simulink model "ModelPWMGenerators"  (R2026a)
settings: Solver=VariableStepAuto  StopTime=2e-4  MaxStep=1e-7
libraries: ConverterLibrary x6
settings Model: Creator=vsolaise  LastModifiedBy=vsolaise

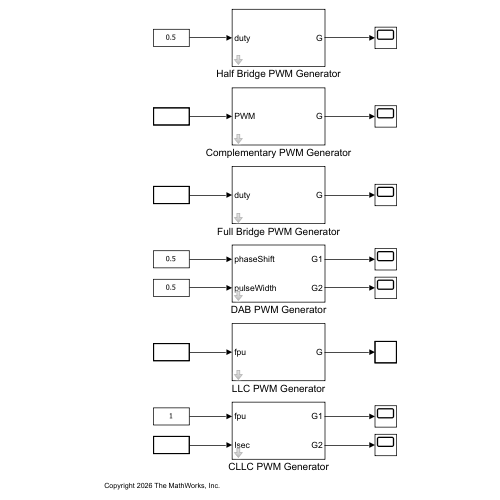
[thumbnail: Simulink's stored preview of the top-level diagram]
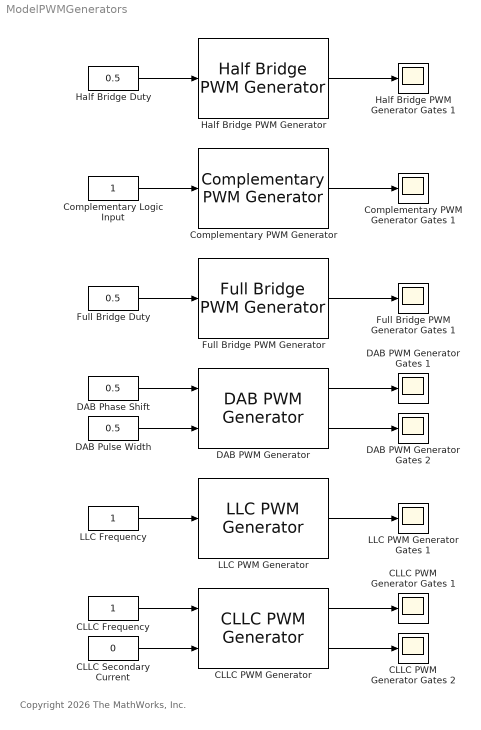
== system ModelPWMGenerators ==
  note: Copyright 2026 The MathWorks, Inc.
  CLLC Frequency : Constant
  CLLC PWM Generator : ConverterLibrary/Controller/PWM Generators/CLLC PWM Generator  solverMode=Variable-step (continuous)  Ts=1e-8  Fbase=100e3  fpuMin=0.6  fpuMax=1.55  pulseWidth=0.5  Tdead=250e-9  Ith=0.5  fpuSrLower=0.97  fpuSrUpper=1.03  Tsr=100e-9  gateVoltageOn=15  gateVoltageOff=0  srGateVoltageOn=15  srGateVoltageOff=0
  CLLC PWM Generator Gates 1 : Scope
  CLLC PWM Generator Gates 2 : Scope
  CLLC Secondary Current : Constant  Value=0
  Complementary Logic Input : Constant
  Complementary PWM Generator : ConverterLibrary/Controller/PWM Generators/Complementary PWM Generator  solverMode=Variable-step (continuous)  Ts=1e-8  Tdead=100e-9  inputLogicThreshold=0.5  gateVoltageOn=15  gateVoltageOff=0
  Complementary PWM Generator Gates 1 : Scope
  DAB PWM Generator : ConverterLibrary/Controller/PWM Generators/DAB PWM Generator  solverMode=Variable-step (continuous)  Ts=1e-8  Fsw=100e3  Tdead=100e-9  primaryGateVoltageOn=15  primaryGateVoltageOff=0  secondaryGateVoltageOn=15  secondaryGateVoltageOff=0
  DAB PWM Generator Gates 1 : Scope
  DAB PWM Generator Gates 2 : Scope
  DAB Phase Shift : Constant  Value=0.5
  DAB Pulse Width : Constant  Value=0.5
  Full Bridge Duty : Constant  Value=0.5
  Full Bridge PWM Generator : ConverterLibrary/Controller/PWM Generators/Full Bridge PWM Generator  solverMode=Variable-step (continuous)  Ts=1e-8  Fsw=100e3  Tdead=100e-9  gateVoltageOn=15  gateVoltageOff=0
  Full Bridge PWM Generator Gates 1 : Scope
  Half Bridge Duty : Constant  Value=0.5
  Half Bridge PWM Generator : ConverterLibrary/Controller/PWM Generators/Half Bridge PWM Generator  solverMode=Variable-step (continuous)  Ts=1e-8  Fsw=100e3  Tdead=100e-9  gateVoltageOn=15  gateVoltageOff=0
  Half Bridge PWM Generator Gates 1 : Scope
  LLC Frequency : Constant
  LLC PWM Generator : ConverterLibrary/Controller/PWM Generators/LLC PWM Generator  solverMode=Variable-step (continuous)  Ts=1e-8  Fbase=100e3  fpuMin=0.5  fpuMax=2  pulseWidth=0.5  Tdead=100e-9  gateVoltageOn=15  gateVoltageOff=0
  LLC PWM Generator Gates 1 : Scope
  wires:
  Half Bridge Duty/1 -> Half Bridge PWM Generator/1
  Half Bridge PWM Generator/1 -> Half Bridge PWM Generator Gates 1/1
  Complementary Logic Input/1 -> Complementary PWM Generator/1
  Complementary PWM Generator/1 -> Complementary PWM Generator Gates 1/1
  Full Bridge Duty/1 -> Full Bridge PWM Generator/1
  Full Bridge PWM Generator/1 -> Full Bridge PWM Generator Gates 1/1
  DAB Phase Shift/1 -> DAB PWM Generator/1
  DAB Pulse Width/1 -> DAB PWM Generator/2
  DAB PWM Generator/1 -> DAB PWM Generator Gates 1/1
  DAB PWM Generator/2 -> DAB PWM Generator Gates 2/1
  LLC Frequency/1 -> LLC PWM Generator/1
  LLC PWM Generator/1 -> LLC PWM Generator Gates 1/1
  CLLC Frequency/1 -> CLLC PWM Generator/1
  CLLC Secondary Current/1 -> CLLC PWM Generator/2
  CLLC PWM Generator/1 -> CLLC PWM Generator Gates 1/1
  CLLC PWM Generator/2 -> CLLC PWM Generator Gates 2/1
